simulink model "servo_laser_test"  (R2025b)
settings: Solver=FixedStepDiscrete  StartTime=0.0  StopTime=inf  FixedStep=0.05  RelTol=1e-3  EnableMultiTasking=on
libraries: raspberrypiBasiclib x2
settings Model: Creator=jeets  LastModifiedBy=jeets
settings SolverCC: PositivePriorityOrder=on
settings DataIOCC: ReturnWorkspaceOutputs=off
settings OptimizationCC: EnhancedBackFolding=on  PassReuseOutputArgsAs=Individual arguments  ZeroExternalMemoryAtStartup=off  ZeroInternalMemoryAtStartup=off  MaxStackSize=200000  OptimizeBlockOrder=speed  DifferentSizesBufferReuse=on  OptimizationCustomize=off  EfficientTunableParamExpr=on
settings DebuggingCC: ParameterTunabilityLossMsg=error
settings HardwareCC: ProdBitPerPointer=32.0  ProdBitPerSizeT=32.0  ProdBitPerPtrDiffT=32.0  ProdLargestAtomicInteger=Long  ProdLargestAtomicFloat=Double  ProdWordSize=32.0  ProdLongLongMode=on  ProdHWDeviceType=ARM Compatible->ARM Cortex-A (32-bit)
settings RTWCC: SystemTargetFile=ert.tlc  HardwareBoard=Raspberry Pi  TLCOptions="-aInlineSetEventsForThisBaseRateFcn=TLC_FALSE -aSuppressMultiTaskScheduler=TLC_FALSE  -aRateBasedStepFcn=0"  TemplateMakefile=ert_default_tmf  Toolchain=GNU GCC Embedded Linux  BuildConfiguration=Faster Runs  Description=Embedded Coder
settings CodeAppCC: ForceParamTrailComments=on  IgnoreCustomStorageClasses=off  OperatorAnnotations=on  SimulinkDataObjDesc=on  SFDataObjDesc=on  InsertBlockDesc=on
settings ERTTargetCC: ExtModeTransport=2.0  ExtModeStaticAlloc=on  ExtModeMexFile=ext_xcp  ExtModeIntrfLevel=Level2 - Open  InlinedParameterPlacement=Hierarchical  CodeReplacementLibrary=ARM Cortex-A CMSIS  SupportVariableSizeSignals=on

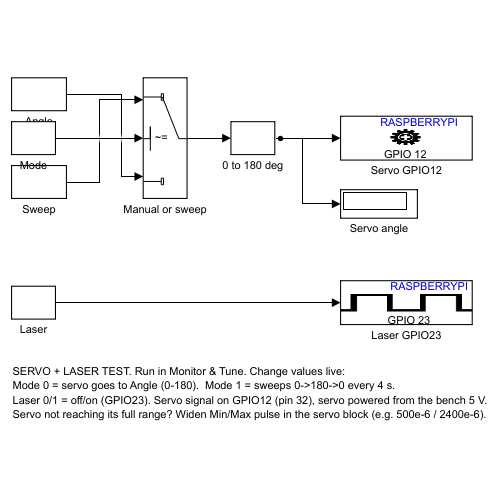
[thumbnail: Simulink's stored preview of the top-level diagram]
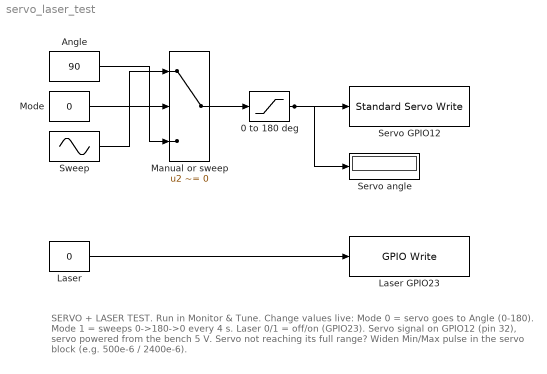
== system servo_laser_test ==
  note: SERVO + LASER TEST. Run in Monitor & Tune. Change values live:
      | Mode 0 = servo goes to Angle (0-180).  Mode 1 = sweeps 0->180->0 every 4 s.
      | Laser 0/1 = off/on (GPIO23). Servo signal on GPIO12 (pin 32), servo powered from the bench 5 V.
      | Servo not reaching its full range? Widen Min/Max pulse in the servo block (e.g. 500e-6 / 2400e-6).
  0 to 180 deg : Saturate  UpperLimit=180  LowerLimit=0
  Angle : Constant  Value=90
  Laser : Constant  Value=0  OutDataTypeStr=boolean
  Laser GPIO23 : raspberrypiBasiclib/GPIO Write  BoardProperty=Pi 3 Model B+  gpio=23  blockPlatform=Raspberry Pi  PinNumber=17  board=[]  direction=[]
  Manual or sweep : Switch  Criteria=u2 ~= 0  SaturateOnIntegerOverflow=off  InputSameDT=off
  Mode : Constant  Value=0
  Servo GPIO12 : raspberrypiBasiclib/Standard Servo Write  board=Pi 3 Model B+  Pin_=12  MinPulseDuration=1000e-6  MaxPulseDuration=2000e-6  blockPlatform=Raspberry Pi
  Servo angle : Display
  Sweep : Sin  Amplitude=90  Bias=90  Frequency=2*pi/4  SampleTime=0.05
  wires:
  Sweep/1 -> Manual or sweep/1
  Mode/1 -> Manual or sweep/2
  Angle/1 -> Manual or sweep/3
  Manual or sweep/1 -> 0 to 180 deg/1
  0 to 180 deg/1 -> Servo GPIO12/1, Servo angle/1
  Laser/1 -> Laser GPIO23/1
